simulink model "Three_Stages"  (R2023a)
settings: Solver=FixedStepDiscrete  StartTime=0.0  StopTime=5000  FixedStep=1  RelTol=1e-3
values from neighbouring files (symbols this model uses):
  fw = zeros(16384, 1, 'uint32')    [test.m]
libraries: hdlsllib x27, simulink x27, etargetslib x1
(part 2 of 5)

== system Three_Stages/LDRB_LDRH ==
  In1 : Inport
  In3 : Inport  Port=2
  read_data : Inport  Port=3
  Bit Slice1 : hdlsllib/Logic and Bit Operations/Bit Slice  lidx=1  ridx=0
  Bit Slice2 : hdlsllib/Logic and Bit Operations/Bit Slice  lidx=31  ridx=16
  Bit Slice3 : hdlsllib/Logic and Bit Operations/Bit Slice  lidx=15  ridx=0
  Bit Slice4 : hdlsllib/Logic and Bit Operations/Bit Slice  lidx=31  ridx=24
  Bit Slice5 : hdlsllib/Logic and Bit Operations/Bit Slice  lidx=23  ridx=16
  Bit Slice6 : hdlsllib/Logic and Bit Operations/Bit Slice  lidx=15  ridx=8
  Bit Slice7 : hdlsllib/Logic and Bit Operations/Bit Slice  lidx=7  ridx=0
  Constant1 : Constant  Value=103  OutDataTypeStr=uint8
  Constant4 : Constant  Value=80  OutDataTypeStr=uint8
  Constant6 : Constant  Value=81  OutDataTypeStr=uint8
  Data Type Conversion{,1,3,5} (4 alike) : DataTypeConversion  OutDataTypeStr=uint32  SaturateOnIntegerOverflow=off  RndMeth=Floor
  Data Type Conversion2 : DataTypeConversion  OutDataTypeStr=int32  SaturateOnIntegerOverflow=off  RndMeth=Floor
  Data Type Conversion4 : DataTypeConversion  OutDataTypeStr=int32  SaturateOnIntegerOverflow=off  RndMeth=Floor
  Equal1 : RelationalOperator  Operator===  OutDataTypeStr=boolean  RndMeth=Simplest  InputSameDT=off
  Equal4 : RelationalOperator  Operator===  OutDataTypeStr=boolean  RndMeth=Simplest  InputSameDT=off
  Equal6 : RelationalOperator  Operator===  OutDataTypeStr=boolean  RndMeth=Simplest  InputSameDT=off
  Extract Bits : simulink/Logic and Bit Operations/Extract Bits  bitsToExtract=Range of bits  numBits=8  bitIdxRange=[1 1]  outScalingMode=Treat bit field as an integer
  Logical Operator : Logic  Operator=OR  AllPortsSameDT=off  OutDataTypeStr=boolean
  Multiport Switch : MultiPortSwitch  DataPortOrder=Zero-based contiguous  Inputs=4  zeroidx=on  SaturateOnIntegerOverflow=off  InputSameDT=off
  Multiport Switch1 : MultiPortSwitch  DataPortOrder=Zero-based contiguous  Inputs=2  zeroidx=on  SaturateOnIntegerOverflow=off  InputSameDT=off
  Shift Arithmetic : ArithShift  BitShiftNumber=24  BitShiftDirection=Left
  Shift Arithmetic1 : ArithShift  BitShiftNumber=24  BitShiftDirection=Right
  Shift Arithmetic2 : ArithShift  BitShiftNumber=16  BitShiftDirection=Left
  Shift Arithmetic3 : ArithShift  BitShiftNumber=16  BitShiftDirection=Right
  Switch : Switch  Criteria=u2 ~= 0  SaturateOnIntegerOverflow=off  InputSameDT=off
  Switch2 : Switch  Criteria=u2 ~= 0  SaturateOnIntegerOverflow=off  InputSameDT=off
  Out1 : Outport
  wires:
  Bit Slice7/1 -> Multiport Switch/2  "byte0[7:0]"
  Bit Slice6/1 -> Multiport Switch/3  "byte1[7:0]"
  Bit Slice5/1 -> Multiport Switch/4  "byte2[7:0]"
  Bit Slice4/1 -> Multiport Switch/5  "byte3[7:0]"
  In1/1 -> Extract Bits/1, Bit Slice1/1  "mem_addr"
  Bit Slice3/1 -> Multiport Switch1/2  "half_lo[15:0]"
  Bit Slice2/1 -> Multiport Switch1/3  "half_hi[15:0]"
  Multiport Switch1/1 -> Data Type Conversion1/1  "sel_half[15:0]"
  Multiport Switch/1 -> Data Type Conversion/1  "sel_byte[7:0]"
  Data Type Conversion/1 -> Switch/1, Shift Arithmetic/1  "zext_byte[31:0]"
  Shift Arithmetic/1 -> Data Type Conversion2/1
  Data Type Conversion2/1 -> Shift Arithmetic1/1
  Shift Arithmetic1/1 -> Data Type Conversion3/1
  Data Type Conversion4/1 -> Shift Arithmetic3/1
  Shift Arithmetic3/1 -> Data Type Conversion5/1
  Data Type Conversion1/1 -> Switch2/1, Shift Arithmetic2/1  "zext_half"
  Shift Arithmetic2/1 -> Data Type Conversion4/1
  Equal4/1 -> Logical Operator/2  "is_ldrb"
  read_data/1 -> Bit Slice6/1, Bit Slice5/1, Bit Slice4/1, Switch/3, Bit Slice2/1, Bit Slice3/1, Bit Slice7/1  "mem_rdata"
  Equal6/1 -> Switch2/2  "is_ldrh"
  Switch/1 -> Switch2/3
  Constant4/1 -> Equal4/2
  Constant6/1 -> Equal6/2
  In3/1 -> Equal1/1, Equal4/1, Equal6/1  "ex_opcode"
  Switch2/1 -> Out1/1  "load_data_selected"
  Bit Slice1/1 -> Multiport Switch/1
  Extract Bits/1 -> Multiport Switch1/1  "control"
  Equal1/1 -> Logical Operator/1  "is_ldrb"
  Constant1/1 -> Equal1/2
  Logical Operator/1 -> Switch/2

== system Three_Stages/LDR_Target ==
  ex_instr_addr : Inport
  Add1 : Sum  OutDataTypeStr=uint32
  Bitwise Operator : simulink/Logic and Bit Operations/Bitwise Operator  logicop=AND  UseBitMask=on  BitMask=0xFFFFFFFC  BitMaskRealWorld=Stored Integer
  Constant4 : Constant  Value=4  OutDataTypeStr=uint32
  ldr_target : Outport
  wires:
  Constant4/1 -> Add1/2
  Add1/1 -> Bitwise Operator/1
  Bitwise Operator/1 -> ldr_target/1  "ldr_target"
  ex_instr_addr/1 -> Add1/1

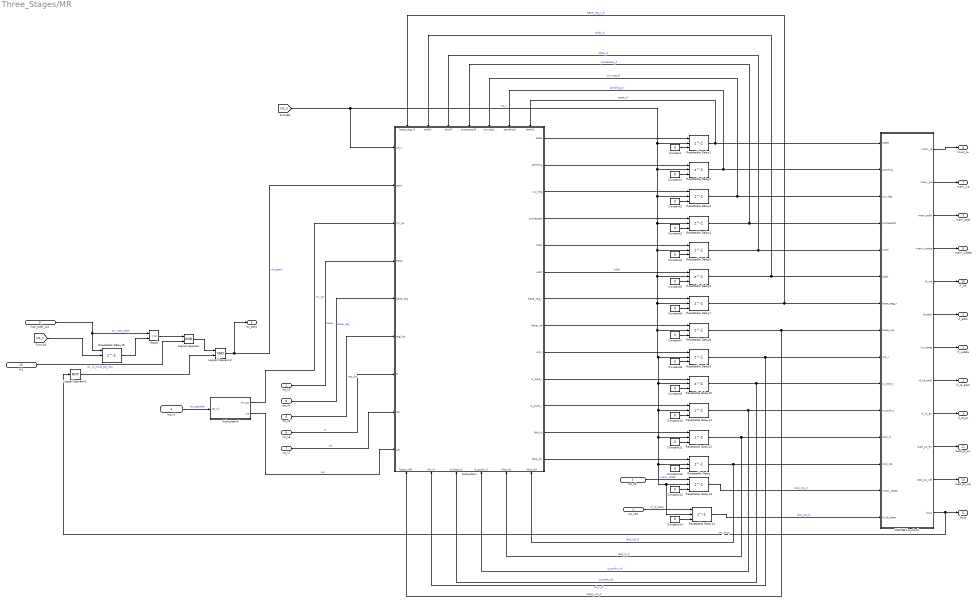
== system Three_Stages/MR ==
  rst_n3 : Inport
  rst_n10 : Inport  Port=2
  rst_n9 : Inport  Port=3  OutDataTypeStr=uint32
  rst_n1 : Inport  Port=4
  instr_addr_out : Inport  Port=5
  rst_n5 : Inport  Port=6
  rst_n7 : Inport  Port=7
  rst_n4 : Inport  Port=8
  rst_n6 : Inport  Port=9
  In1 : Inport  Port=10
  Constant{,2..4,6,11..12} (7 alike) : Constant  Value=0  OutDataTypeStr=uint8
  Constant1 : Constant  Value=0  OutDataTypeStr=uint16
  Constant10 : Constant  Value=0  OutDataTypeStr=boolean
  Constant{5,7,13..14} (4 alike) : Constant  Value=0  OutDataTypeStr=uint32
  Constant8 : Constant  Value=0  OutDataTypeStr=boolean
  Constant9 : Constant  Value=0  OutDataTypeStr=boolean
  Equal : RelationalOperator  Operator=~=  OutDataTypeStr=boolean  RndMeth=Simplest  InputSameDT=off
  Logical Operator : Logic  AllPortsSameDT=off  OutDataTypeStr=boolean
  Logical Operator1 : Logic  Operator=NOT  AllPortsSameDT=off  OutDataTypeStr=boolean
  Logical Operator2 : Logic  AllPortsSameDT=off  OutDataTypeStr=boolean
  MATLAB Function1 : MATLAB Function  TreatAsAtomicUnit=on
  Resettable Delay{,1..15} (16 alike) : Delay  DelayLength=1  InitialConditionSource=Input port  ExternalReset=Falling
      settings: InputPortMap=u0,r5,p4
  Subsystem : Subsystem
      settings: PortSchema="{\"entries\":[{\"content\":{\"sides\":[{\"content\":{\"connectorIds\":[\"In1\",\"In2\",\"In3\",\"In4\",\"In5\",\"In6\",\"In7\",\"In8\",\"In9\"]},\"type\":\"ConnectorPlacement.EquallySpacedRectSide\",\"uuid\":\"18cec05c-2bb3-4bac-bc09-28dbd3e98bf9\"},{\"content\":{\"connectorIds\":[\"Out1\",\"Out2\",\"Out3\",\"Out4\",\"Out5\",\"Out6\",\"Out7\",\"Out8\",\"Out9\",\"Out10\",\"Out11\",\"Out12\",\"Out13\"],\"side\":\"RIGHT\"},\"type\":\"ConnectorPlacement.EquallySpacedRectSide\",\"uuid\":\"58e6d276-578a-4a6f-87ac-3b0855bd0a82\"},{\"content\":{\"connectorIds\":[\"In10\",\"In11\",\"In12\",\"In13\",\"In14\",\"In15\",\"In16\"],\"side\":\"TOP\"},\"type\":\"ConnectorPlacement.EquallySpacedRectSide\",\"uuid\":\"a00e333a-b3d3-443b-9423-a2553426b111\"},{\"content\":{\"connectorIds\":[\"In17\",\"In18\",\"In19\",\"In20\",\"In21\",\"In22\"],\"side\":\"BOTTOM\"},\"type\":\"ConnectorPlacement.EquallySpacedRectSide\",\"uuid\":\"7f7bed57-1a93-4a44-b29c-2cfc6cbcba11\"}]},\"type\":\"ConnectorPlacement.EquallySpacedConnector\",\"uuid\":\"48a416f6-ecda-4738-a4db-dfc888de9068\"}],\"packageUris\":[\"http://schema.mathworks.com/mf0/Connector/R2020b\"],\"version\":\"1.0\"}"
  Subsystem6 : Subsystem
  rf_addr : Outport  OutDataTypeStr=uint8
  rf_wdata : Outport  Port=2
  rf_rd_addr : Outport  Port=3
  rf_rd_en : Outport  Port=4
  mr_start : Outport  Port=5
  mem_wdata : Outport  Port=6
  mem_we : Outport  Port=7
  mem_re : Outport  Port=8
  mem_addr : Outport  Port=9  OutDataTypeStr=uint32
  rf_we : Outport  Port=10
  busy : Outport  Port=11
  load_pc_en : Outport  Port=12
  load_pc_val : Outport  Port=13
  wires:
  [rst_n] -> Subsystem/1(rst_n), Resettable Delay14/2, Resettable Delay13/2, Resettable Delay/2, Resettable Delay12/2, Resettable Delay11/2, Resettable Delay10/2, Resettable Delay9/2, Resettable Delay8/2, Resettable Delay7/2, Resettable Delay6/2, Resettable Delay5/2, Resettable Delay4/2, Resettable Delay3/2, Resettable Delay2/2, Resettable Delay1/2  "rst_n"
  Resettable Delay1/1 -> MATLAB Function1/1(state), Subsystem/16(state1)  "state_d"
  Resettable Delay2/1 -> MATLAB Function1/2(pending), Subsystem/15(pending1)  "pending_d"
  Resettable Delay3/1 -> MATLAB Function1/3(cur_reg), Subsystem/14(cur_reg1)  "cur_reg_d"
  Resettable Delay4/1 -> MATLAB Function1/4(processed), Subsystem/13(processed1)  "processed_d"
  Resettable Delay5/1 -> MATLAB Function1/5(total), Subsystem/12(total1)  "total_d"
  Resettable Delay8/1 -> MATLAB Function1/8(base_val), Subsystem/17(base_val1)  "base_val_d"
  Resettable Delay7/1 -> MATLAB Function1/7(base_reg_r), Subsystem/10(base_reg_r1)  "base_reg_r_d"
  Resettable Delay6/1 -> MATLAB Function1/6(addr), Subsystem/11(addr1)  "addr_d"
  Resettable Delay9/1 -> MATLAB Function1/9(wb_r), Subsystem/18(wb_r1)  "wb_r_d"
  Resettable Delay12/1 -> Subsystem/21(ldrd_rt1), MATLAB Function1/12(ldrd_rt)  "ldrd_rt_d"
  Resettable Delay11/1 -> Subsystem/20(is_push_r1), MATLAB Function1/11(is_push_r)  "is_push_r_d"
  Resettable Delay10/1 -> MATLAB Function1/10(is_load_r), Subsystem/19(is_load_r1)  "is_load_r_d"
  Resettable Delay/1 -> Subsystem/22(ldrd_rt3), MATLAB Function1/13(ldrd_rt2)  "ldrd_rt2_d"
  MATLAB Function1/11(load_pc_val) -> load_pc_val/1
  MATLAB Function1/7(rf_wdata) -> rf_wdata/1
  MATLAB Function1/8(rf_rd_addr) -> rf_rd_addr/1
  MATLAB Function1/4(mem_wdata) -> mem_wdata/1
  MATLAB Function1/9(rf_rd_en) -> rf_rd_en/1
  MATLAB Function1/2(mem_we) -> mem_we/1
  MATLAB Function1/1(mem_re) -> mem_re/1
  MATLAB Function1/5(rf_we) -> rf_we/1
  MATLAB Function1/6(rf_addr) -> rf_addr/1
  MATLAB Function1/10(load_pc_en) -> load_pc_en/1
  MATLAB Function1/3(mem_addr) -> mem_addr/1
  Constant/1 -> Resettable Delay1/3
  Constant1/1 -> Resettable Delay2/3
  Constant2/1 -> Resettable Delay3/3
  Constant3/1 -> Resettable Delay4/3
  Constant4/1 -> Resettable Delay5/3
  Constant5/1 -> Resettable Delay6/3
  Constant6/1 -> Resettable Delay7/3
  Constant7/1 -> Resettable Delay8/3
  Constant8/1 -> Resettable Delay9/3
  Constant9/1 -> Resettable Delay10/3
  Constant10/1 -> Resettable Delay11/3
  Constant11/1 -> Resettable Delay12/3
  Constant12/1 -> Resettable Delay/3
  rst_n9/1 -> Resettable Delay13/1  "mem_rdata"
  rst_n10/1 -> Resettable Delay14/1  "rf_rd_data"
  Subsystem6/1(mr_op) -> Subsystem/3(mr_op)  "mr_op"
  rst_n3/1 -> Subsystem/4(base)  "base"
  rst_n4/1 -> Subsystem/5(base_reg)  "base_reg"
  rst_n5/1 -> Subsystem/6(reg_list)  "reg_list"
  rst_n6/1 -> Subsystem/7(rt)  "rt"
  rst_n7/1 -> Subsystem/8(rt2)  "rt2"
  Subsystem6/2(wb) -> Subsystem/9(wb)  "wb"
  Subsystem/1(state) -> Resettable Delay1/1
  Subsystem/2(pending) -> Resettable Delay2/1
  Subsystem/3(cur_reg) -> Resettable Delay3/1
  Subsystem/4(processed) -> Resettable Delay4/1
  Subsystem/5(total) -> Resettable Delay5/1
  Subsystem/6(addr) -> Resettable Delay6/1  "addr"
  Subsystem/7(base_reg_r) -> Resettable Delay7/1
  Subsystem/8(base_val) -> Resettable Delay8/1
  Subsystem/9(wb_r) -> Resettable Delay9/1
  Subsystem/10(is_load_r) -> Resettable Delay10/1
  Subsystem/11(is_push_r) -> Resettable Delay11/1
  Subsystem/12(ldrd_rt) -> Resettable Delay12/1
  Subsystem/13(ldrd_rt2) -> Resettable Delay/1
  Resettable Delay13/1 -> MATLAB Function1/14(mem_rdata)  "ldrd_rt2_d"
  Resettable Delay14/1 -> MATLAB Function1/15(rf_rd_data)  "ldrd_rt2_d"
  Constant13/1 -> Resettable Delay13/3
  Constant14/1 -> Resettable Delay14/3
  In1/1 -> Logical Operator/2  "ex_is_multi_op_raw"
  Logical Operator2/1 -> mr_start/1, Subsystem/2(start)  "mr_start"
  Equal/1 -> Logical Operator/1
  instr_addr_out/1 -> Equal/1, Resettable Delay15/1  "ex_instr_addr"
  [rst_n] -> Resettable Delay15/2
  Logical Operator/1 -> Logical Operator2/1
  MATLAB Function1/12(busy) -> Logical Operator1/1, busy/1  "mr_busy"
  Logical Operator1/1 -> Logical Operator2/2
  Resettable Delay15/1 -> Equal/2
  rst_n1/1 -> Subsystem6/1(rst_n1)  "ex_opcode"

== system Three_Stages/PC ==
  In1 : Inport
  In2 : Inport  Port=2
  In4 : Inport  Port=3
  In5 : Inport  Port=4
  In6 : Inport  Port=5
  Resettable Delay : Delay  DelayLength=1  InitialConditionSource=Input port  ExternalReset=Falling
      settings: InputPortMap=u0,r5,p4
  Switch : Switch  Criteria=u2 ~= 0  SaturateOnIntegerOverflow=off  InputSameDT=off
  Switch1 : Switch  Criteria=u2 ~= 0  SaturateOnIntegerOverflow=off  InputSameDT=off
  Out1 : Outport  OutDataTypeStr=uint32
  wires:
  In6/1 -> Resettable Delay/3  "init_pc"
  Switch1/1 -> Resettable Delay/1
  Switch/1 -> Switch1/3
  In5/1 -> Switch1/1  "flush_target"
  Resettable Delay/1 -> Switch/1, Out1/1  "instr_addr"
  In2/1 -> Switch/2  "stall"
  In1/1 -> Switch/3  "next_instr"
  In4/1 -> Switch1/2  "flush"
  [rst_n] -> Resettable Delay/2  "rst_n"

== system Three_Stages/Prefetch_Unit ==
  In2 : Inport
  instr_data : Inport  Port=2  OutDataTypeStr=uint32
  instr_data2 : Inport  Port=3
  instr_data3 : Inport  Port=4
  instr_data4 : Inport  Port=5
  Constant : Constant  Value=zeros(8,1,'uint16')
  Constant1 : Constant  Value=0  OutDataTypeStr=uint8
  Constant2 : Constant  Value=0  OutDataTypeStr=uint8
  Constant3 : Constant  Value=0  OutDataTypeStr=uint8
  Constant4 : Constant  Value=0  OutDataTypeStr=uint32
  Constant5 : Constant  Value=0  OutDataTypeStr=boolean
  Constant6 : Constant  Value=0  OutDataTypeStr=boolean
  Resettable Delay{,1..7} (8 alike) : Delay  DelayLength=1  InitialConditionSource=Input port  ExternalReset=Falling
      settings: InputPortMap=u0,r5,p4
  Subsystem : Subsystem
      settings: PortSchema="{\"entries\":[{\"content\":{\"sides\":[{\"content\":{\"connectorIds\":[\"In1\",\"In2\",\"In3\",\"In4\"]},\"type\":\"ConnectorPlacement.EquallySpacedRectSide\",\"uuid\":\"6a41aa12-c6ed-4179-803d-49044b936052\"},{\"content\":{\"connectorIds\":[\"Out1\",\"Out2\",\"Out3\",\"Out4\",\"Out5\",\"Out6\",\"Out7\",\"Out8\"],\"side\":\"RIGHT\"},\"type\":\"ConnectorPlacement.EquallySpacedRectSide\",\"uuid\":\"8907858c-80bb-4ba2-aed8-2e664f4798ff\"},{\"content\":{\"connectorIds\":[\"In5\",\"In6\",\"In7\",\"In8\"],\"side\":\"TOP\"},\"type\":\"ConnectorPlacement.EquallySpacedRectSide\",\"uuid\":\"d385d123-5e68-4d44-82a6-b4662cc99c7b\"},{\"content\":{\"connectorIds\":[\"In9\",\"In10\",\"In11\",\"In12\"],\"side\":\"BOTTOM\"},\"type\":\"ConnectorPlacement.EquallySpacedRectSide\",\"uuid\":\"83c7c30f-cef9-40bc-8916-19f66b971374\"}]},\"type\":\"ConnectorPlacement.EquallySpacedConnector\",\"uuid\":\"a169f654-665e-4fd7-8819-89c58e46c9a3\"}],\"packageUris\":[\"http://schema.mathworks.com/mf0/Connector/R2020b\"],\"version\":\"1.0\"}"
  Out1 : Outport
  Out2 : Outport  Port=2
  Out3 : Outport  Port=3
  Out4 : Outport  Port=4
  wires:
  [rst_n] -> Resettable Delay2/2, Resettable Delay7/2, Resettable Delay6/2, Resettable Delay5/2, Resettable Delay4/2, Resettable Delay3/2, Resettable Delay1/2, Resettable Delay/2  "rst_n"
  Constant/1 -> Resettable Delay/3
  Constant1/1 -> Resettable Delay1/3
  In2/1 -> Resettable Delay4/3  "IF_PC"
  Constant4/1 -> Resettable Delay5/3
  Constant5/1 -> Resettable Delay6/3
  Constant6/1 -> Resettable Delay7/3
  Constant3/1 -> Resettable Delay3/3
  Constant2/1 -> Resettable Delay2/3
  Subsystem/1(next_fifo_mem) -> Resettable Delay/1
  Subsystem/2(next_wr_ptr) -> Resettable Delay1/1
  Subsystem/3(next_rd_ptr) -> Resettable Delay2/1
  Subsystem/4(next_count) -> Resettable Delay3/1
  Subsystem/5(next_fetch_pc) -> Resettable Delay4/1
  Subsystem/6(next_instr) -> Resettable Delay5/1
  Subsystem/7(next_instr_width) -> Resettable Delay6/1
  Subsystem/8(next_pop_valid) -> Resettable Delay7/1
  Resettable Delay7/1 -> Out4/1, Subsystem/12(pop_valid)  "pop_valid"
  Resettable Delay6/1 -> Out3/1, Subsystem/11(instr_width)  "instr_width"
  Resettable Delay5/1 -> Out2/1, Subsystem/10(instr)  "instr"
  Resettable Delay4/1 -> Out1/1, Subsystem/9(fetch_pc)  "fetch_pc"
  Resettable Delay1/1 -> Subsystem/7(wr_ptr)
  Resettable Delay2/1 -> Subsystem/6(rd_ptr)
  Resettable Delay3/1 -> Subsystem/5(count)
  instr_data/1 -> Subsystem/1(instr_data)  "instr_data"
  instr_data2/1 -> Subsystem/2(flush)  "flush"
  instr_data3/1 -> Subsystem/3(flush_target)  "flush_target"
  instr_data4/1 -> Subsystem/4(stall)  "stall"
  Resettable Delay/1 -> Subsystem/8(fifo_mem)

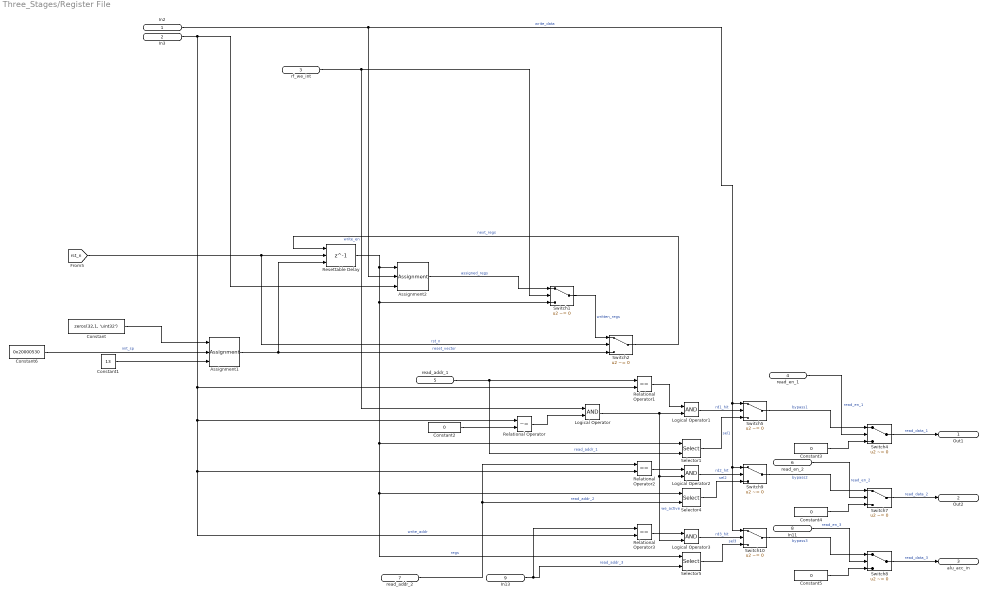
== system Three_Stages/Register File ==
  In2 : Inport  OutDataTypeStr=uint32
  In3 : Inport  Port=2  OutDataTypeStr=uint32
  rf_we_int : Inport  Port=3  OutDataTypeStr=boolean
  read_en_1 : Inport  Port=4  OutDataTypeStr=boolean
  read_addr_1 : Inport  Port=5  OutDataTypeStr=uint8
  read_en_2 : Inport  Port=6  OutDataTypeStr=boolean
  read_addr_2 : Inport  Port=7  OutDataTypeStr=uint8
  In11 : Inport  Port=8  OutDataTypeStr=boolean
  In13 : Inport  Port=9  OutDataTypeStr=uint8
  Assignment1 : Assignment  IndexMode=Zero-based  DiagnosticForDimensions=Warning  IndexOptions=Index vector (port)  Indices=1  OutputSizes=1  RuntimeRangeChecks=on
  Assignment2 : Assignment  IndexMode=Zero-based  DiagnosticForDimensions=Warning  IndexOptions=Index vector (port)  Indices=1  OutputSizes=1  RuntimeRangeChecks=on
  Constant : Constant  Value=zeros(32,1, 'uint32')  OutDataTypeStr=uint32  LockScale=on
  Constant1 : Constant  Value=13  OutDataTypeStr=uint32
  Constant{2..5} (4 alike) : Constant  Value=0  OutDataTypeStr=uint32  LockScale=on
  Constant6 : Constant  Value=0x20000530
  Logical Operator{,1..3} (4 alike) : Logic  AllPortsSameDT=off  OutDataTypeStr=boolean
  Relational Operator : RelationalOperator  Operator=~=  OutDataTypeStr=boolean  RndMeth=Simplest  InputSameDT=off
  Relational Operator1 : RelationalOperator  Operator===  OutDataTypeStr=boolean  RndMeth=Simplest  InputSameDT=off
  Relational Operator2 : RelationalOperator  Operator===  OutDataTypeStr=boolean  RndMeth=Simplest  InputSameDT=off
  Relational Operator3 : RelationalOperator  Operator===  OutDataTypeStr=boolean  RndMeth=Simplest  InputSameDT=off
  Resettable Delay : Delay  DelayLength=1  InitialConditionSource=Input port  ExternalReset=Falling
      settings: InputPortMap=u0,r5,p4
  Selector1 : Selector  IndexMode=Zero-based  IndexOptions=Index vector (port)  Indices=[1 3]  OutputSizes=1
  Selector4 : Selector  IndexMode=Zero-based  IndexOptions=Index vector (port)  Indices=[1 3]  OutputSizes=1
  Selector5 : Selector  IndexMode=Zero-based  IndexOptions=Index vector (port)  Indices=[1 3]  OutputSizes=1
  Switch{1..2,4..5,7..10} (8 alike) : Switch  Criteria=u2 ~= 0  OutDataTypeStr=uint32  SaturateOnIntegerOverflow=off  InputSameDT=off
  Out1 : Outport
  Out2 : Outport  Port=2
  alu_acc_in : Outport  Port=3
  wires:
  Constant2/1 -> Relational Operator/2
  Selector4/1 -> Switch9/3  "sel2"
  In3/1 -> Relational Operator3/2, Relational Operator2/2, Relational Operator/1, Relational Operator1/2, Assignment2/3  "write_addr"
  Selector1/1 -> Switch5/3  "sel1"
  Constant3/1 -> Switch4/3
  Assignment1/1 -> Switch2/3, Resettable Delay/3  "reset_vector"
  Constant1/1 -> Assignment1/3
  Resettable Delay/1 -> Selector5/1, Selector4/1, Selector1/1, Switch1/3, Assignment2/1  "regs"
  [rst_n] -> Switch2/2, Resettable Delay/2  "rst_n"
  Logical Operator1/1 -> Switch5/2  "rd1_hit"
  Constant4/1 -> Switch7/3
  Switch7/1 -> Out2/1  "read_data_2"
  Relational Operator3/1 -> Logical Operator3/1
  Switch10/1 -> Switch8/1  "bypass3"
  In2/1 -> Switch10/1, Switch9/1, Switch5/1, Assignment2/2  "write_data"
  Relational Operator/1 -> Logical Operator/2
  Constant6/1 -> Assignment1/2  "init_sp"
  read_addr_1/1 -> Relational Operator1/1, Selector1/2  "read_addr_1"
  Logical Operator2/1 -> Switch9/2  "rd2_hit"
  Switch5/1 -> Switch4/1  "bypass1"
  Constant/1 -> Assignment1/1
  Logical Operator3/1 -> Switch10/2  "rd3_hit"
  Switch9/1 -> Switch7/1  "bypass2"
  Constant5/1 -> Switch8/3
  Logical Operator/1 -> Logical Operator1/2, Logical Operator3/2, Logical Operator2/2  "we_active"
  Relational Operator2/1 -> Logical Operator2/1
  Switch1/1 -> Switch2/1  "written_regs"
  Selector5/1 -> Switch10/3  "sel3"
  Relational Operator1/1 -> Logical Operator1/1
  Assignment2/1 -> Switch1/1  "assigned_regs"
  In13/1 -> Selector5/2, Relational Operator3/1  "read_addr_3"
  read_en_1/1 -> Switch4/2  "read_en_1"
  Switch4/1 -> Out1/1  "read_data_1"
  read_addr_2/1 -> Selector4/2, Relational Operator2/1  "read_addr_2"
  Switch8/1 -> alu_acc_in/1  "read_data_3"
  Switch2/1 -> Resettable Delay/1  "next_regs"
  rf_we_int/1 -> Switch1/2, Logical Operator/1  "write_en"
  In11/1 -> Switch8/2  "read_en_3"
  read_en_2/1 -> Switch7/2  "read_en_2"

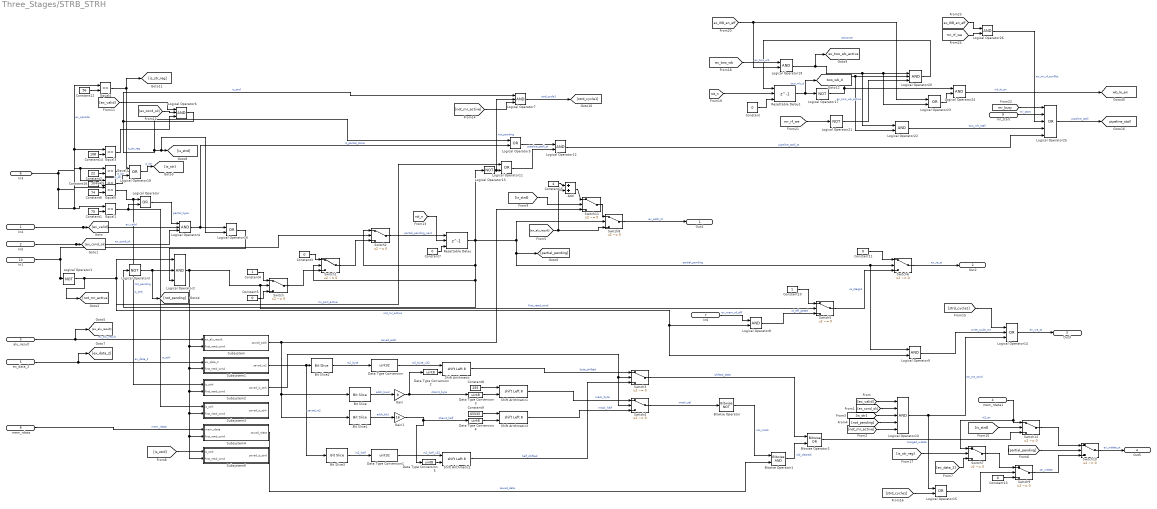
== system Three_Stages/STRB_STRH ==
  In4 : Inport
  In5 : Inport  Port=2
  alu_result : Inport  Port=3
  mem_rdata1 : Inport  Port=4
  ex_data_2 : Inport  Port=5
  In3 : Inport  Port=6
  In6 : Inport  Port=7
  mem_rdata : Inport  Port=8
  mr_start : Inport  Port=9
  In1 : Inport  Port=10
  Add : Sum
  Bit Slice : hdlsllib/Logic and Bit Operations/Bit Slice  lidx=1  ridx=0
  Bit Slice1 : hdlsllib/Logic and Bit Operations/Bit Slice  lidx=1  ridx=1
  Bit Slice2 : hdlsllib/Logic and Bit Operations/Bit Slice  lidx=7  ridx=0
  Bit Slice3 : hdlsllib/Logic and Bit Operations/Bit Slice  lidx=15  ridx=0
  Bitwise Operator : simulink/Logic and Bit Operations/Bitwise Operator  logicop=NOT  UseBitMask=off  BitMask=bin2dec('11011001')  BitMaskRealWorld=Stored Integer
  Bitwise Operator1 : simulink/Logic and Bit Operations/Bitwise Operator  logicop=AND  UseBitMask=off  NumInputPorts=2  BitMask=bin2dec('11011001')  BitMaskRealWorld=Stored Integer
  Bitwise Operator2 : simulink/Logic and Bit Operations/Bitwise Operator  logicop=OR  UseBitMask=off  NumInputPorts=2  BitMask=bin2dec('11011001')  BitMaskRealWorld=Stored Integer
  Constant : Constant  Value=0  OutDataTypeStr=boolean
  Constant1 : Constant  Value=75  OutDataTypeStr=uint8
  Constant10 : Constant  OutDataTypeStr=uint8
  Constant{3,5,7,11} (4 alike) : Constant  Value=0  OutDataTypeStr=uint8
  Constant12 : Constant  Value=56  OutDataTypeStr=uint8
  Constant13 : Constant  Value=0  OutDataTypeStr=uint32
  Constant14 : Constant  Value=108  OutDataTypeStr=uint8
  Constant15 : Constant  Value=4  OutDataTypeStr=uint8
  Constant16 : Constant  Value=76  OutDataTypeStr=uint8
  Constant2 : Constant  Value=22  OutDataTypeStr=uint8
  Constant4 : Constant  OutDataTypeStr=uint8
  Constant6 : Constant  Value=74  OutDataTypeStr=uint8
  Constant8 : Constant  Value=255  OutDataTypeStr=uint32
  Constant9 : Constant  Value=65535  OutDataTypeStr=uint32
  Data Type Conversion : DataTypeConversion  OutDataTypeStr=uint32  SaturateOnIntegerOverflow=off  RndMeth=Floor
  Data Type Conversion1 : DataTypeConversion  OutDataTypeStr=uint32  SaturateOnIntegerOverflow=off  RndMeth=Floor
  Data Type Conversion{2..5} (4 alike) : DataTypeConversion  OutDataTypeStr=uint8  SaturateOnIntegerOverflow=off  RndMeth=Floor
  Equal{1..6} (6 alike) : RelationalOperator  Operator===  OutDataTypeStr=boolean  RndMeth=Simplest  InputSameDT=off
  Gain : Gain  Gain=8
  Gain1 : Gain  Gain=16
  Logical Operator{,5,11,15..16,23} (6 alike) : Logic  Operator=OR  AllPortsSameDT=off  OutDataTypeStr=boolean
  Logical Operator{1,3,13,17,21} (5 alike) : Logic  Operator=NOT  AllPortsSameDT=off  OutDataTypeStr=boolean
  Logical Operator10 : Logic  Inputs=5  AllPortsSameDT=off  OutDataTypeStr=boolean
  Logical Operator{8..9,12,19,22,24,26} (7 alike) : Logic  AllPortsSameDT=off  OutDataTypeStr=boolean
  Logical Operator14 : Logic  Operator=OR  Inputs=3  AllPortsSameDT=off  OutDataTypeStr=boolean
  Logical Operator18 : Logic  Operator=OR  Inputs=3  AllPortsSameDT=off  OutDataTypeStr=boolean
  Logical Operator{2,4,6..7,20} (5 alike) : Logic  Inputs=3  AllPortsSameDT=off  OutDataTypeStr=boolean
  Logical Operator25 : Logic  Operator=OR  Inputs=5  AllPortsSameDT=off  OutDataTypeStr=boolean
  Resettable Delay : Delay  DelayLength=1  InitialConditionSource=Input port  ExternalReset=Falling
      settings: InputPortMap=u0,r5,p4
  Resettable Delay1 : Delay  DelayLength=1  InitialConditionSource=Input port  ExternalReset=Falling
      settings: InputPortMap=u0,r5,p4
  Shift Arithmetic{,1..3} (4 alike) : ArithShift  BitShiftNumberSource=Input port  BitShiftNumber=8  BitShiftDirection=Left
      settings: InputPortMap=u0,p1
  Subsystem : Subsystem
  Subsystem1 : Subsystem
  Subsystem2 : Subsystem
  Subsystem3 : Subsystem
  Subsystem4 : Subsystem
  Subsystem6 : Subsystem
  Switch{,1..12} (13 alike) : Switch  Criteria=u2 ~= 0  SaturateOnIntegerOverflow=off  InputSameDT=off
  Out4 : Outport
  Out2 : Outport  Port=2
  Out3 : Outport  Port=3
  Out5 : Outport  Port=4
  tag scope: ex_two_wb_active=global, pipeline_stall=global, two_wb_d=global, wb_lo_en=global
  wires:
  Constant6/1 -> Equal6/2
  In3/1 -> Equal1/1, Equal6/1, Equal5/1, Equal2/1, Equal4/1, Equal3/1  "ex_opcode"
  Constant1/1 -> Equal1/2
  Logical Operator4/1 -> Logical Operator5/2, Logical Operator16/1  "is_partial_store"
  Constant2/1 -> Equal2/2
  Logical Operator18/1 -> [is_str]  "is_str"
  Logical Operator1/1 -> Logical Operator2/1, Logical Operator9/2, Logical Operator8/2, [not_mr_active]  "not_mr_active"
  Logical Operator3/1 -> [not_pending], Logical Operator2/2  "not_pending"
  In4/1 -> [ex_valid], Logical Operator4/2  "ex_valid"
  In5/1 -> [ex_cond_ok], Logical Operator4/3  "ex_cond_ok"
  Logical Operator/1 -> Logical Operator4/1  "partial_type"
  Switch/1 -> Switch1/3
  Switch1/1 -> Switch2/3
  In1/1 -> Logical Operator11/1, Logical Operator1/1, Switch2/2  "mr_port_active"
  Resettable Delay/1 -> Switch2/1, Switch1/2, Logical Operator3/1, Logical Operator13/1, [partial_pending], Logical Operator9/1, Switch6/2, Switch8/2  "partial_pending"
  Constant3/1 -> Switch1/1
  Constant4/1 -> Switch/1
  Constant5/1 -> Switch/3
  Switch2/1 -> Resettable Delay/1  "partial_pending_next"
  Logical Operator2/1 -> Subsystem6/2(first_read_cond), Subsystem4/2(first_read_cond), Subsystem3/2(first_read_cond), Subsystem2/2(first_read_cond), Subsystem1/2(first_read_cond), Subsystem/2(first_read_cond), Switch5/2, Switch/2  "first_read_cond"
  ex_data_2/1 -> [ex_data_2], Subsystem1/1(ex_data_2)  "ex_data_2"
  Equal6/1 -> Subsystem2/1(is_strb), Logical Operator/1  "is_strb"
  Equal1/1 -> Subsystem3/1(is_strh), Logical Operator/2  "is_strh"
  mem_rdata/1 -> Subsystem4/1(mem_rdata)  "mem_rdata"
  Constant7/1 -> Resettable Delay/3
  [rst_n] -> Resettable Delay/2
  alu_result/1 -> [ex_alu_result], Subsystem/1(ex_alu_result)  "ex_alu_result"
  Bit Slice/1 -> Gain/1  "addr_low2"
  Subsystem/1(saved_addr) -> Switch11/3, Bit Slice1/1, Bit Slice/1  "saved_addr"
  Bit Slice1/1 -> Gain1/1  "addr_bit1"
  Gain/1 -> Data Type Conversion3/1, Data Type Conversion2/1  "shamt_byte"
  Gain1/1 -> Data Type Conversion5/1, Data Type Conversion4/1  "shamt_half"
  Subsystem1/1(saved_rs2) -> Bit Slice3/1, Bit Slice2/1  "saved_rs2"
  Bit Slice2/1 -> Data Type Conversion/1  "rs2_byte"
  Data Type Conversion/1 -> Shift Arithmetic/1  "rs2_byte_u32"
  Constant8/1 -> Shift Arithmetic1/1
  Bit Slice3/1 -> Data Type Conversion1/1  "rs2_half"
  Data Type Conversion1/1 -> Shift Arithmetic2/1  "rs2_half_u32"
  Shift Arithmetic2/1 -> Switch3/3  "half_shifted"
  Constant9/1 -> Shift Arithmetic3/1
  Subsystem2/1(saved_is_strb) -> Switch4/2, Switch3/2
  Switch3/1 -> Bitwise Operator2/1  "shifted_data"
  Switch4/1 -> Bitwise Operator/1  "mask_sel"
  Shift Arithmetic/1 -> Switch3/1  "byte_shifted"
  Shift Arithmetic1/1 -> Switch4/1  "mask_byte"
  Shift Arithmetic3/1 -> Switch4/3  "mask_half"
  Bitwise Operator/1 -> Bitwise Operator1/1  "not_mask"
  Subsystem4/1(saved_rdata) -> Bitwise Operator1/2  "saved_data"
  Bitwise Operator1/1 -> Bitwise Operator2/2  "old_cleared"
  Bitwise Operator2/1 -> Switch12/3  "merged_wdata"
  In6/1 -> Logical Operator8/1  "ex_mem_rd_eff"
  Logical Operator8/1 -> Switch5/3  "rd_eff_gated"
  Constant10/1 -> Switch5/1
  Constant11/1 -> Switch6/1
  Switch5/1 -> Switch6/3  "re_stage1"
  Switch6/1 -> Out2/1  "ex_re_st"
  Logical Operator9/1 -> Logical Operator14/2  "write_cycle_we"
  [ex_valid] -> Logical Operator10/1
  [ex_cond_ok] -> Logical Operator10/2
  [is_str] -> Logical Operator10/3
  [not_mr_active] -> Logical Operator10/5
  [not_pending] -> Logical Operator10/4
  Logical Operator10/1 -> Logical Operator14/3, Logical Operator15/1  "str_we_cond"
  Logical Operator14/1 -> Out3/1  "ex_we_st"
  [ex_alu_result] -> Add/2, Switch8/3
  Switch8/1 -> Out4/1  "ex_addr_st"
  Switch9/1 -> Switch10/3  "str_wdata"
  Switch10/1 -> Out5/1  "ex_wdata_st"
  [partial_pending] -> Switch10/2
  Constant13/1 -> Switch9/3
  [ex_data_2] -> Switch7/3
  Logical Operator11/1 -> Logical Operator12/2  "pipeline_stall_st"
  Data Type Conversion2/1 -> Shift Arithmetic/2
  Data Type Conversion3/1 -> Shift Arithmetic1/2
  Data Type Conversion4/1 -> Shift Arithmetic3/2
  Data Type Conversion5/1 -> Shift Arithmetic2/2
  Logical Operator13/1 -> Logical Operator7/2, Logical Operator11/2  "not_pending"
  Logical Operator12/1 -> Logical Operator25/5  "pipeline_stall_st"
  Constant14/1 -> Equal3/2
  Logical Operator6/1 -> Logical Operator16/2, [is_strd], Logical Operator5/1, Logical Operator7/1  "is_strd"
  Logical Operator5/1 -> Logical Operator12/1
  [is_strd] -> Subsystem6/1(is_strd)
  Switch11/1 -> Switch8/1
  [is_strd] -> Switch11/2
  Add/1 -> Switch11/1
  Constant15/1 -> Add/1
  Switch12/1 -> Switch10/1
  mem_rdata1/1 -> Switch12/1, Switch7/1  "rt2_ex"
  [ex_valid] -> Logical Operator6/1
  [ex_cond_ok] -> Logical Operator6/2
  Equal3/1 -> Logical Operator6/3
  [not_mr_active] -> Logical Operator7/3
  Logical Operator7/1 -> [strd_cycle1]  "strd_cycle1"
  [strd_cycle1] -> Logical Operator14/1
  [strd_cycle1] -> Logical Operator15/2
  Logical Operator15/1 -> Switch9/2
  Logical Operator16/1 -> Logical Operator2/3
  [is_strd] -> Switch12/2
  Constant12/1 -> Equal4/2
  Equal4/1 -> Logical Operator18/1, [is_str_reg]  "is_str_reg"
  Equal2/1 -> Logical Operator18/2  "is_str"
  Switch7/1 -> Switch9/1
  [is_str_reg] -> Switch7/2
  mr_start/1 -> Logical Operator25/2  "mr_start"
  Logical Operator26/1 -> Logical Operator25/3  "ex_mr_rf_conflict"
  Logical Operator25/1 -> [pipeline_stall]  "pipeline_stall"
  [mr_busy] -> Logical Operator25/1
  Logical Operator24/1 -> [wb_lo_en]  "wb_lo_en"
  Logical Operator23/1 -> Logical Operator24/2
  Logical Operator22/1 -> Logical Operator25/4  "two_wb_stall"
  Logical Operator20/1 -> Resettable Delay1/1  "advance"
  [mr_rf_we] -> Logical Operator21/1
  Logical Operator21/1 -> Logical Operator20/3
  Logical Operator17/1 -> Logical Operator22/2, Logical Operator20/2, Logical Operator24/1
  [rst_n] -> Resettable Delay1/2
  Logical Operator19/1 -> [ex_two_wb_active], Logical Operator22/1, Logical Operator23/2, Logical Operator20/1  "ex_two_wb_active"
  [ex_WB_en_eff] -> Logical Operator19/2, Logical Operator23/1
  Constant/1 -> Resettable Delay1/3
  Resettable Delay1/1 -> [two_wb_d], Logical Operator17/1  "two_wb_d"
  [ex_two_wb] -> Logical Operator19/1  "ex_two_wb"
  [ex_WB_en_eff] -> Logical Operator26/1
  [mr_rf_we] -> Logical Operator26/2
  Equal5/1 -> Logical Operator18/3  "is_str"
  Constant16/1 -> Equal5/2

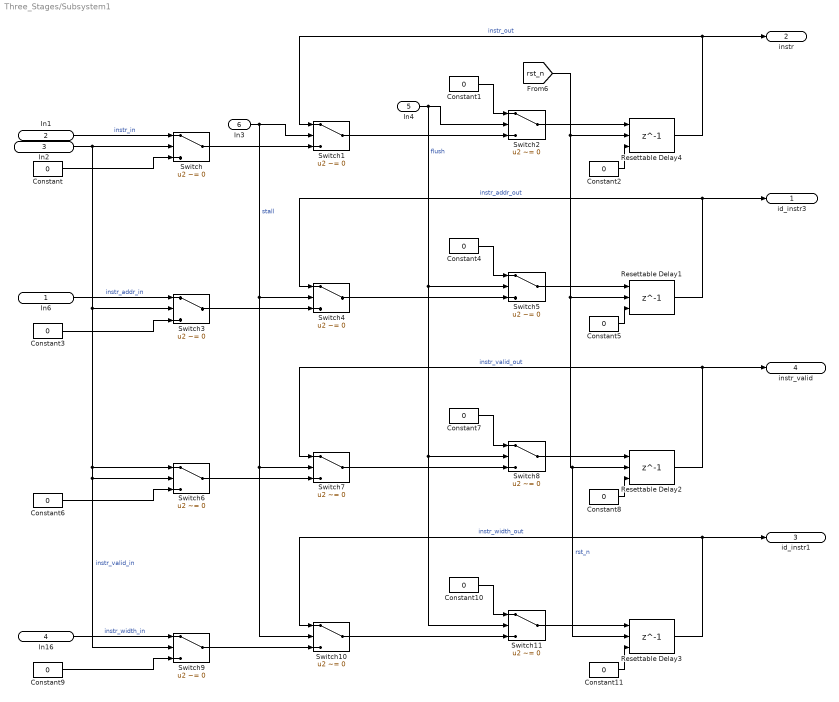
== system Three_Stages/Subsystem1 ==
  In6 : Inport
  In1 : Inport  Port=2
  In2 : Inport  Port=3  OutDataTypeStr=boolean
  In16 : Inport  Port=4
  In4 : Inport  Port=5  OutDataTypeStr=boolean
  In3 : Inport  Port=6  OutDataTypeStr=boolean
  Constant{,1..11} (12 alike) : Constant  Value=0  OutDataTypeStr=uint32
  Resettable Delay{1..4} (4 alike) : Delay  DelayLength=1  InitialConditionSource=Input port  ExternalReset=Falling
      settings: InputPortMap=u0,r5,p4
  Switch{,1..11} (12 alike) : Switch  Criteria=u2 ~= 0  SaturateOnIntegerOverflow=off  InputSameDT=off
  id_instr3 : Outport
  instr : Outport  Port=2
  id_instr1 : Outport  Port=3
  instr_valid : Outport  Port=4
  wires:
  In6/1 -> Switch3/1  "instr_addr_in"
  In3/1 -> Switch10/2, Switch7/2, Switch4/2, Switch1/2  "stall"
  Switch5/1 -> Resettable Delay1/1
  Switch11/1 -> Resettable Delay3/1
  Switch8/1 -> Resettable Delay2/1
  Resettable Delay2/1 -> instr_valid/1, Switch7/1  "instr_valid_out"
  Constant8/1 -> Resettable Delay2/3
  In16/1 -> Switch9/1  "instr_width_in"
  Constant6/1 -> Switch6/3
  Switch3/1 -> Switch4/3
  In2/1 -> Switch6/1, Switch6/2, Switch9/2, Switch3/2, Switch/2  "instr_valid_in"
  Switch6/1 -> Switch7/3
  Switch7/1 -> Switch8/3
  Constant7/1 -> Switch8/1
  Switch/1 -> Switch1/3
  Constant3/1 -> Switch3/3
  [rst_n] -> Resettable Delay3/2, Resettable Delay2/2, Resettable Delay1/2, Resettable Delay4/2  "rst_n"
  Constant/1 -> Switch/3
  In4/1 -> Switch11/2, Switch8/2, Switch5/2, Switch2/2  "flush"
  Switch1/1 -> Switch2/3
  Resettable Delay1/1 -> id_instr3/1, Switch4/1  "instr_addr_out"
  Resettable Delay4/1 -> instr/1, Switch1/1  "instr_out"
  Switch4/1 -> Switch5/3
  Switch10/1 -> Switch11/3
  Resettable Delay3/1 -> id_instr1/1, Switch10/1  "instr_width_out"
  Constant4/1 -> Switch5/1
  Constant1/1 -> Switch2/1
  Constant5/1 -> Resettable Delay1/3
  Constant2/1 -> Resettable Delay4/3
  Constant10/1 -> Switch11/1
  In1/1 -> Switch/1  "instr_in"
  Switch2/1 -> Resettable Delay4/1
  Constant9/1 -> Switch9/3
  Constant11/1 -> Resettable Delay3/3
  Switch9/1 -> Switch10/3

== system Three_Stages/Subsystem13 ==
  data_2_out : Inport
  alu_src_b_out : Inport  Port=2
  alu_shamt_out : Inport  Port=3
  alu_shamt_out1 : Inport  Port=4
  alu_shamt_out2 : Inport  Port=5
  Constant : Constant  Value=0
  Constant1 : Constant  Value=11
  Constant2 : Constant  Value=13
  Constant3 : Constant  Value=15
  Constant4 : Constant  Value=29
  Constant5 : Constant  Value=0
  Constant6 : Constant  Value=31
  Logical Operator3 : Logic  Operator=OR  Inputs=5  AllPortsSameDT=off  OutDataTypeStr=boolean
  Logical Operator4 : Logic  Operator=NOT  Inputs=4  AllPortsSameDT=off  OutDataTypeStr=boolean
  Logical Operator5 : Logic  Inputs=3  AllPortsSameDT=off  OutDataTypeStr=boolean
  Relational Operator{1..5,7} (6 alike) : RelationalOperator  Operator===  OutDataTypeStr=boolean  RndMeth=Simplest  InputSameDT=off
  Relational Operator6 : RelationalOperator  Operator=>  OutDataTypeStr=boolean  RndMeth=Simplest  InputSameDT=off
  Shift Arithmetic : ArithShift  BitShiftNumberSource=Input port  BitShiftNumber=8  BitShiftDirection=Left
      settings: InputPortMap=u0,p1
  Shift Arithmetic1 : ArithShift  BitShiftNumberSource=Input port  BitShiftNumber=8  BitShiftDirection=Right
      settings: InputPortMap=u0,p1
  Switch1 : Switch  Criteria=u2 ~= 0  SaturateOnIntegerOverflow=off  InputSameDT=off
  Switch4 : Switch  Criteria=u2 ~= 0  SaturateOnIntegerOverflow=off  InputSameDT=off
  Out1 : Outport
  wires:
  Shift Arithmetic/1 -> Switch1/3
  Switch4/1 -> Out1/1  "alu_b"
  alu_shamt_out/1 -> Relational Operator6/1, Shift Arithmetic1/2, Shift Arithmetic/2  "ex_alu_shamt"
  data_2_out/1 -> Shift Arithmetic1/1, Switch4/3, Shift Arithmetic/1  "ex_data_2"
  alu_src_b_out/1 -> Relational Operator5/2  "alu_src_b_out"
  Relational Operator5/1 -> Logical Operator5/2
  Constant/1 -> Relational Operator6/2
  Relational Operator6/1 -> Logical Operator5/3
  Constant1/1 -> Relational Operator1/2
  Constant2/1 -> Relational Operator2/2
  alu_shamt_out1/1 -> Relational Operator7/1, Relational Operator4/1, Relational Operator3/1, Relational Operator2/1, Relational Operator1/1
  Relational Operator2/1 -> Logical Operator3/2  "LSR"
  Relational Operator1/1 -> Logical Operator3/1  "LSL"
  Shift Arithmetic1/1 -> Switch1/1
  alu_shamt_out2/1 -> Switch1/2  "ex_alu_shift_type"
  Switch1/1 -> Switch4/1  "shifted"
  Constant3/1 -> Relational Operator3/2
  Relational Operator3/1 -> Logical Operator3/3  "ASR.W"
  Constant4/1 -> Relational Operator4/2
  Relational Operator4/1 -> Logical Operator3/4  "ROR.W"
  Logical Operator3/1 -> Logical Operator4/1
  Logical Operator4/1 -> Logical Operator5/1  "is_not_shift"
  Logical Operator5/1 -> Switch4/2
  Constant5/1 -> Relational Operator5/1
  Constant6/1 -> Relational Operator7/2
  Relational Operator7/1 -> Logical Operator3/5  "UBFX"

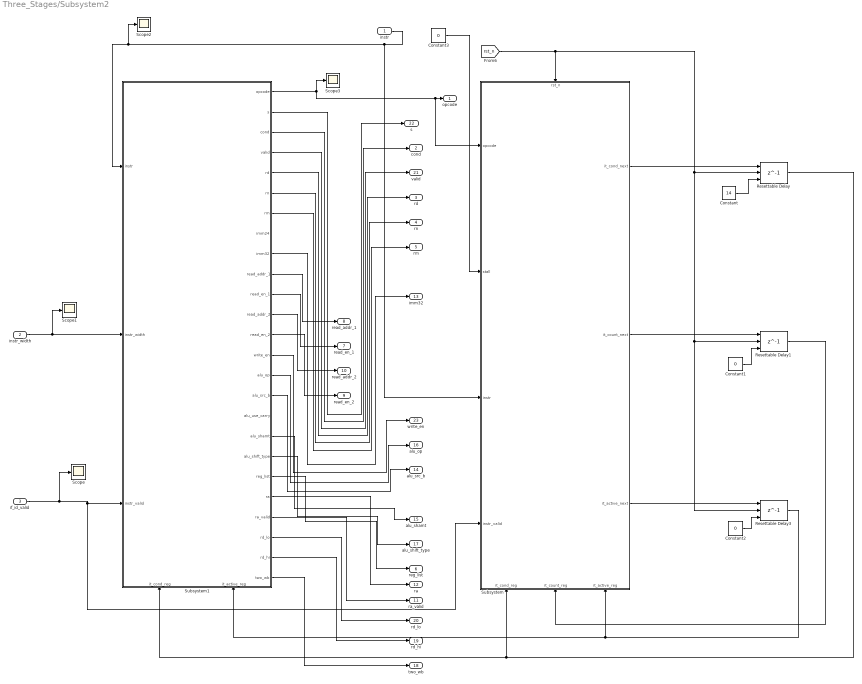
== system Three_Stages/Subsystem2 ==
  instr : Inport
  instr_width : Inport  Port=2  OutDataTypeStr=boolean
  if_id_valid : Inport  Port=3  OutDataTypeStr=boolean
  Constant : Constant  Value=14  OutDataTypeStr=uint8
  Constant1 : Constant  Value=0  OutDataTypeStr=uint8
  Constant2 : Constant  Value=0  OutDataTypeStr=boolean
  Constant3 : Constant  Value=0  OutDataTypeStr=boolean
  Resettable Delay : Delay  DelayLength=1  InitialConditionSource=Input port  ExternalReset=Falling
      settings: InputPortMap=u0,r5,p4
  Resettable Delay1 : Delay  DelayLength=1  InitialConditionSource=Input port  ExternalReset=Falling
      settings: InputPortMap=u0,r5,p4
  Resettable Delay3 : Delay  DelayLength=1  InitialConditionSource=Input port  ExternalReset=Falling
      settings: InputPortMap=u0,r5,p4
  Scope{,1..3} (4 alike) : Scope
  Subsystem : Subsystem
      settings: PortSchema="{\"entries\":[{\"content\":{\"sides\":[{\"content\":{\"connectorIds\":[\"In1\",\"In2\",\"In3\",\"In4\"]},\"type\":\"ConnectorPlacement.EquallySpacedRectSide\",\"uuid\":\"317e3dad-cb1a-43c4-b47f-58f87d7e043e\"},{\"content\":{\"connectorIds\":[\"Out1\",\"Out2\",\"Out3\"],\"side\":\"RIGHT\"},\"type\":\"ConnectorPlacement.EquallySpacedRectSide\",\"uuid\":\"12791d8d-2277-406c-bd16-0c13a6e4b681\"},{\"content\":{\"connectorIds\":[\"In5\"],\"side\":\"TOP\"},\"type\":\"ConnectorPlacement.EquallySpacedRectSide\",\"uuid\":\"45c96fa8-41a8-4cd0-8976-1116a2bdd932\"},{\"content\":{\"connectorIds\":[\"In6\",\"In7\",\"In8\"],\"side\":\"BOTTOM\"},\"type\":\"ConnectorPlacement.EquallySpacedRectSide\",\"uuid\":\"892b2249-487d-4897-befd-edcd812cbb9f\"}]},\"type\":\"ConnectorPlacement.EquallySpacedConnector\",\"uuid\":\"2f25677e-f182-4579-8db9-213c5f4ee455\"}],\"packageUris\":[\"http://schema.mathworks.com/mf0/Connector/R2020b\"],\"version\":\"1.0\"}"
  Subsystem1 : Subsystem
      settings: PortSchema="{\"entries\":[{\"content\":{\"sides\":[{\"content\":{\"connectorIds\":[\"In1\",\"In2\",\"In3\"]},\"type\":\"ConnectorPlacement.EquallySpacedRectSide\",\"uuid\":\"06c131a9-ff48-4f57-8b36-9c8f6f9fb960\"},{\"content\":{\"connectorIds\":[\"Out1\",\"Out2\",\"Out3\",\"Out4\",\"Out5\",\"Out6\",\"Out7\",\"Out8\",\"Out9\",\"Out10\",\"Out11\",\"Out12\",\"Out13\",\"Out14\",\"Out15\",\"Out16\",\"Out17\",\"Out18\",\"Out19\",\"Out20\",\"Out21\",\"Out22\",\"Out23\",\"Out24\",\"Out25\"],\"side\":\"RIGHT\"},\"type\":\"ConnectorPlacement.EquallySpacedRectSide\",\"uuid\":\"30117597-05bd-414d-a263-fe3296f4d102\"},{\"content\":{\"side\":\"TOP\"},\"type\":\"ConnectorPlacement.EquallySpacedRectSide\",\"uuid\":\"dcff9dee-4d39-4452-a406-510372c26920\"},{\"content\":{\"connectorIds\":[\"In4\",\"In5\"],\"side\":\"BOTTOM\"},\"type\":\"ConnectorPlacement.EquallySpacedRectSide\",\"uuid\":\"1f797825-3e9e-489d-accc-0e8fd6c126ea\"}]},\"type\":\"ConnectorPlacement.EquallySpacedConnector\",\"uuid\":\"164a078c-82a8-4695-9150-66eb237dee78\"}],\"packageUris\":[\"http://schema.mathworks.com/mf0/Connector/R2020b\"],\"version\":\"1.0\"}"
  opcode : Outport  OutDataTypeStr=uint8
  cond : Outport  Port=2  OutDataTypeStr=uint8
  rd : Outport  Port=3
  rn : Outport  Port=4
  rm : Outport  Port=5
  reg_list : Outport  Port=6
  read_en_1 : Outport  Port=7
  read_addr_1 : Outport  Port=8  OutDataTypeStr=uint8
  read_en_2 : Outport  Port=9
  read_addr_2 : Outport  Port=10
  ra_valid : Outport  Port=11
  ra : Outport  Port=12
  imm32 : Outport  Port=13
  alu_src_b : Outport  Port=14
  alu_shamt : Outport  Port=15  OutDataTypeStr=uint8
  alu_op : Outport  Port=16  OutDataTypeStr=uint8
  alu_shift_type : Outport  Port=17
  two_wb : Outport  Port=18
  rd_hi : Outport  Port=19
  rd_lo : Outport  Port=20
  valid : Outport  Port=21
  s : Outport  Port=22  OutDataTypeStr=boolean
  write_en : Outport  Port=23
  wires:
  instr_width/1 -> Scope1/1, Subsystem1/2(instr_width)
  Subsystem1/15(alu_op) -> alu_op/1
  Subsystem1/7(rm) -> rm/1
  Subsystem1/4(valid) -> valid/1
  Subsystem1/3(cond) -> cond/1
  Subsystem1/9(imm32) -> imm32/1
  Subsystem1/14(write_en) -> write_en/1
  Subsystem1/20(reg_list) -> reg_list/1
  Subsystem1/18(alu_shamt) -> alu_shamt/1
  Constant3/1 -> Subsystem/2(stall)
  Subsystem1/6(rn) -> rn/1
  Subsystem1/16(alu_src_b) -> alu_src_b/1
  instr/1 -> Subsystem/3(instr), Scope2/1, Subsystem1/1(instr)
  Subsystem1/2(s) -> s/1
  Subsystem1/5(rd) -> rd/1
  if_id_valid/1 -> Scope/1, Subsystem/4(instr_valid), Subsystem1/3(instr_valid)
  Subsystem1/13(read_en_2) -> read_en_2/1
  Subsystem1/12(read_addr_2) -> read_addr_2/1
  Subsystem1/10(read_addr_1) -> read_addr_1/1
  Subsystem1/19(alu_shift_type) -> alu_shift_type/1
  Subsystem1/11(read_en_1) -> read_en_1/1
  Subsystem/2(it_count_next) -> Resettable Delay1/1
  Subsystem/1(it_cond_next) -> Resettable Delay/1
  [rst_n] -> Subsystem/5(rst_n), Resettable Delay3/2, Resettable Delay1/2, Resettable Delay/2
  Subsystem/3(it_active_next) -> Resettable Delay3/1
  Constant/1 -> Resettable Delay/3
  Constant1/1 -> Resettable Delay1/3
  Constant2/1 -> Resettable Delay3/3
  Resettable Delay3/1 -> Subsystem1/5(it_active_reg), Subsystem/8(it_active_reg)
  Resettable Delay1/1 -> Subsystem/7(it_count_reg)
  Resettable Delay/1 -> Subsystem1/4(it_cond_reg), Subsystem/6(it_cond_reg)
  Subsystem1/1(opcode) -> opcode/1, Subsystem/1(opcode), Scope3/1
  Subsystem1/21(ra) -> ra/1
  Subsystem1/22(ra_valid) -> ra_valid/1
  Subsystem1/23(rd_lo) -> rd_lo/1
  Subsystem1/24(rd_hi) -> rd_hi/1
  Subsystem1/25(two_wb) -> two_wb/1

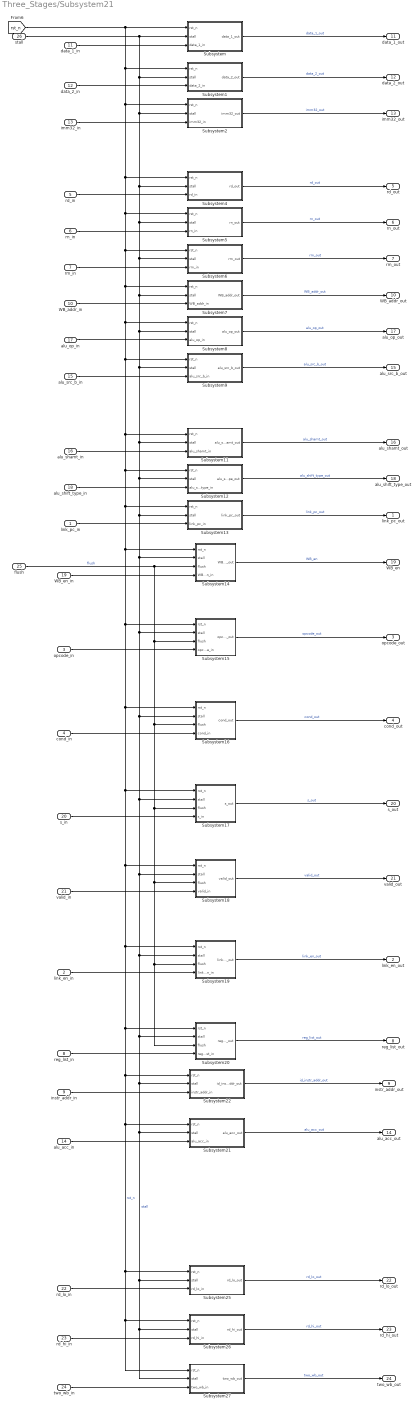
== system Three_Stages/Subsystem21 ==
  link_pc_in : Inport
  link_en_in : Inport  Port=2
  opcode_in : Inport  Port=3
  cond_in : Inport  Port=4
  rd_in : Inport  Port=5
  rn_in : Inport  Port=6
  rm_in : Inport  Port=7
  reg_list_in : Inport  Port=8
  instr_addr_in : Inport  Port=9
  WB_addr_in : Inport  Port=10
  data_1_in : Inport  Port=11
  data_2_in : Inport  Port=12
  imm32_in : Inport  Port=13
  alu_acc_in : Inport  Port=14
  alu_src_b_in : Inport  Port=15
  alu_shamt_in : Inport  Port=16
  alu_op_in : Inport  Port=17
  alu_shift_type_in : Inport  Port=18
  WB_en_in : Inport  Port=19
  s_in : Inport  Port=20
  valid_in : Inport  Port=21
  rd_lo_in : Inport  Port=22
  rd_hi_in : Inport  Port=23
  two_wb_in : Inport  Port=24
  flush : Inport  Port=25  OutDataTypeStr=boolean
  stall : Inport  Port=26  OutDataTypeStr=boolean
  Subsystem : Subsystem
  Subsystem1 : Subsystem
  Subsystem11 : Subsystem
  Subsystem12 : Subsystem
  Subsystem13 : Subsystem
  Subsystem14 : Subsystem
  Subsystem15 : Subsystem
  Subsystem16 : Subsystem
  Subsystem17 : Subsystem
  Subsystem18 : Subsystem
  Subsystem19 : Subsystem
  Subsystem2 : Subsystem
  Subsystem20 : Subsystem
  Subsystem21 : Subsystem
  Subsystem22 : Subsystem
  Subsystem25 : Subsystem
  Subsystem26 : Subsystem
  Subsystem27 : Subsystem
  Subsystem4 : Subsystem
  Subsystem5 : Subsystem
  Subsystem6 : Subsystem
  Subsystem7 : Subsystem
  Subsystem8 : Subsystem
  Subsystem9 : Subsystem
  link_pc_out : Outport
  link_en_out : Outport  Port=2
  opcode_out : Outport  Port=3
  cond_out : Outport  Port=4
  rd_out : Outport  Port=5
  rn_out : Outport  Port=6
  rm_out : Outport  Port=7
  reg_list_out : Outport  Port=8
  instr_addr_out : Outport  Port=9  OutDataTypeStr=uint32
  WB_addr_out : Outport  Port=10
  data_1_out : Outport  Port=11
  data_2_out : Outport  Port=12  OutDataTypeStr=uint32
  imm32_out : Outport  Port=13
  alu_acc_out : Outport  Port=14  OutDataTypeStr=uint32
  alu_src_b_out : Outport  Port=15
  alu_shamt_out : Outport  Port=16
  alu_op_out : Outport  Port=17
  alu_shift_type_out : Outport  Port=18
  WB_en : Outport  Port=19
  s_out : Outport  Port=20
  valid_out : Outport  Port=21
  rd_lo_out : Outport  Port=22  OutDataTypeStr=uint32
  rd_hi_out : Outport  Port=23  OutDataTypeStr=uint32
  two_wb_out : Outport  Port=24  OutDataTypeStr=uint32
  wires:
  Subsystem6/1(rm_out) -> rm_out/1  "rm_out"
  Subsystem13/1(link_pc_out) -> link_pc_out/1  "link_pc_out"
  Subsystem17/1(s_out) -> s_out/1  "s_out"
  flush/1 -> Subsystem20/3(flush), Subsystem19/3(flush), Subsystem18/3(flush), Subsystem17/3(flush), Subsystem16/3(flush), Subsystem15/3(flush), Subsystem14/3(flush)  "flush"
  Subsystem4/1(rd_out) -> rd_out/1  "rd_out"
  alu_src_b_in/1 -> Subsystem9/3(alu_src_b_in)
  Subsystem18/1(valid_out) -> valid_out/1  "valid_out"
  WB_en_in/1 -> Subsystem14/4(WB_en_in)
  alu_shift_type_in/1 -> Subsystem12/3(alu_shift_type_in)
  reg_list_in/1 -> Subsystem20/4(reg_list_in)
  data_2_in/1 -> Subsystem1/3(data_2_in)
  rn_in/1 -> Subsystem5/3(rn_in)
  Subsystem19/1(link_en_out) -> link_en_out/1  "link_en_out"
  s_in/1 -> Subsystem17/4(s_in)
  link_en_in/1 -> Subsystem19/4(link_en_in)
  Subsystem15/1(opcode_out) -> opcode_out/1  "opcode_out"
  opcode_in/1 -> Subsystem15/4(opcode_in)
  data_1_in/1 -> Subsystem/3(data_1_in)
  Subsystem7/1(WB_addr_out) -> WB_addr_out/1  "WB_addr_out"
  Subsystem/1(data_1_out) -> data_1_out/1  "data_1_out"
  Subsystem12/1(alu_shift_type_out) -> alu_shift_type_out/1  "alu_shift_type_out"
  rd_in/1 -> Subsystem4/3(rd_in)
  Subsystem5/1(rn_out) -> rn_out/1  "rn_out"
  link_pc_in/1 -> Subsystem13/3(link_pc_in)
  alu_shamt_in/1 -> Subsystem11/3(alu_shamt_in)
  Subsystem11/1(alu_shamt_out) -> alu_shamt_out/1  "alu_shamt_out"
  imm32_in/1 -> Subsystem2/3(imm32_in)
  alu_op_in/1 -> Subsystem8/3(alu_op_in)
  cond_in/1 -> Subsystem16/4(cond_in)
  Subsystem2/1(imm32_out) -> imm32_out/1  "imm32_out"
  Subsystem8/1(alu_op_out) -> alu_op_out/1  "alu_op_out"
  WB_addr_in/1 -> Subsystem7/3(WB_addr_in)
  Subsystem9/1(alu_src_b_out) -> alu_src_b_out/1  "alu_src_b_out"
  rm_in/1 -> Subsystem6/3(rm_in)
  Subsystem16/1(cond_out) -> cond_out/1  "cond_out"
  Subsystem14/1(WB_en_out) -> WB_en/1  "WB_en"
  Subsystem1/1(data_2_out) -> data_2_out/1  "data_2_out"
  valid_in/1 -> Subsystem18/4(valid_in)
  Subsystem20/1(reg_list_out) -> reg_list_out/1  "reg_list_out"
  instr_addr_in/1 -> Subsystem22/3(instr_addr_in)
  Subsystem22/1(id_instr_addr_out) -> instr_addr_out/1  "id_instr_addr_out"
  Subsystem21/1(alu_acc_out) -> alu_acc_out/1  "alu_acc_out"
  alu_acc_in/1 -> Subsystem21/3(alu_acc_in)
  stall/1 -> Subsystem27/2(stall), Subsystem26/2(stall), Subsystem25/2(stall), Subsystem21/2(stall), Subsystem22/2(stall), Subsystem20/2(stall), Subsystem19/2(stall), Subsystem18/2(stall), Subsystem17/2(stall), Subsystem16/2(stall), Subsystem15/2(stall), Subsystem14/2(stall), Subsystem13/2(stall), Subsystem12/2(stall), Subsystem11/2(stall), Subsystem9/2(stall), Subsystem8/2(stall), Subsystem7/2(stall), Subsystem6/2(stall), Subsystem5/2(stall), Subsystem4/2(stall), Subsystem2/2(stall), Subsystem1/2(stall), Subsystem/2(stall)  "stall"
  [rst_n] -> Subsystem27/1(rst_n), Subsystem26/1(rst_n), Subsystem25/1(rst_n), Subsystem21/1(rst_n), Subsystem22/1(rst_n), Subsystem20/1(rst_n), Subsystem19/1(rst_n), Subsystem18/1(rst_n), Subsystem17/1(rst_n), Subsystem16/1(rst_n), Subsystem15/1(rst_n), Subsystem14/1(rst_n), Subsystem13/1(rst_n), Subsystem12/1(rst_n), Subsystem11/1(rst_n), Subsystem9/1(rst_n), Subsystem8/1(rst_n), Subsystem7/1(rst_n), Subsystem6/1(rst_n), Subsystem5/1(rst_n), Subsystem4/1(rst_n), Subsystem2/1(rst_n), Subsystem1/1(rst_n), Subsystem/1(rst_n)  "rst_n"
  two_wb_in/1 -> Subsystem27/3(two_wb_in)
  rd_hi_in/1 -> Subsystem26/3(rd_hi_in)
  rd_lo_in/1 -> Subsystem25/3(rd_lo_in)
  Subsystem27/1(two_wb_out) -> two_wb_out/1  "two_wb_out"
  Subsystem26/1(rd_hi_out) -> rd_hi_out/1  "rd_hi_out"
  Subsystem25/1(rd_lo_out) -> rd_lo_out/1  "rd_lo_out"

== system Three_Stages/Subsystem3 ==
  ex_opcode : Inport
  is_load_op : Subsystem
  is_multi_load_op : Subsystem
  is_multi_store_op : Subsystem
  is_store_op : Subsystem
  ex_is_load : Outport
  ex_is_store : Outport  Port=2
  ex_is_multi_ld : Outport  Port=3
  ex_is_multi_st : Outport  Port=4
  tag scope: ex_is_load=global, ex_is_store=global
  wires:
  ex_opcode/1 -> is_multi_store_op/1(opcode_out), is_multi_load_op/1(opcode_out), is_store_op/1(opcode_out), is_load_op/1(opcode_out)
  is_store_op/1(Out1) -> [ex_is_store], ex_is_store/1  "ex_is_store"
  is_multi_load_op/1(Out1) -> ex_is_multi_ld/1  "ex_is_multi_ld"
  is_load_op/1(Out1) -> [ex_is_load], ex_is_load/1  "ex_is_load"
  is_multi_store_op/1(Out1) -> ex_is_multi_st/1  "ex_is_multi_st"

== system Three_Stages/Subsystem4 ==
  Logical Operator12 : Logic  Inputs=3  AllPortsSameDT=off  OutDataTypeStr=boolean
  Logical Operator14 : Logic  Operator=NOT  AllPortsSameDT=off  OutDataTypeStr=boolean
  Logical Operator20 : Logic  Operator=NOT  AllPortsSameDT=off  OutDataTypeStr=boolean
  Subsystem3 : Subsystem
      settings: PortSchema="{\"entries\":[{\"content\":{\"sides\":[{\"content\":{\"connectorIds\":[\"In1\"]},\"type\":\"ConnectorPlacement.EquallySpacedRectSide\",\"uuid\":\"40573664-4769-4fb7-9c63-c2f7966a6555\"},{\"content\":{\"connectorIds\":[\"Out1\"],\"side\":\"RIGHT\"},\"type\":\"ConnectorPlacement.EquallySpacedRectSide\",\"uuid\":\"c1a8e94e-7852-4aa5-80e4-70f14ab388f1\"},{\"content\":{\"connectorIds\":[\"In2\"],\"side\":\"TOP\"},\"type\":\"ConnectorPlacement.EquallySpacedRectSide\",\"uuid\":\"5825a1fb-6959-466e-8f29-436bda723f2d\"}]},\"type\":\"ConnectorPlacement.EquallySpacedConnector\",\"uuid\":\"859313ab-9182-495f-b704-a5cbe29d3b19\"}],\"packageUris\":[\"http://schema.mathworks.com/mf0/Connector/R2020b\"],\"version\":\"1.0\"}"
  Out1 : Outport
  wires:
  [rst_n] -> Subsystem3/2(In2)
  Subsystem3/1(Out1) -> Logical Operator20/1  "flush_apsr_d"
  Logical Operator12/1 -> Out1/1
  Logical Operator14/1 -> Logical Operator12/2
  [ex_valid_eff] -> Logical Operator12/1
  Logical Operator20/1 -> Logical Operator12/3
  [flush] -> Subsystem3/1(In1)
  [ex_is_multi_op] -> Logical Operator14/1
